simulink model "AFC_FFNN_trainscg_15_15_15_15_15_Nor_July_15_RepCont"  (R2021a)
settings: Solver=ode15s  StartTime=0.0  StopTime=T  MaxStep=.01  RelTol=1e-3
InitFcn:
  | ensure_patch_sig_in();
undefined symbols (not defined in the file): AF_sensor_tol, fault_time, fuel_inj_tol, kappa_tol, MAF_sensor_tol, pump_tol, tau_ww_tol, x_gain, x_offset, y_gain, y_offset
libraries: neural x82
(part 3 of 4)

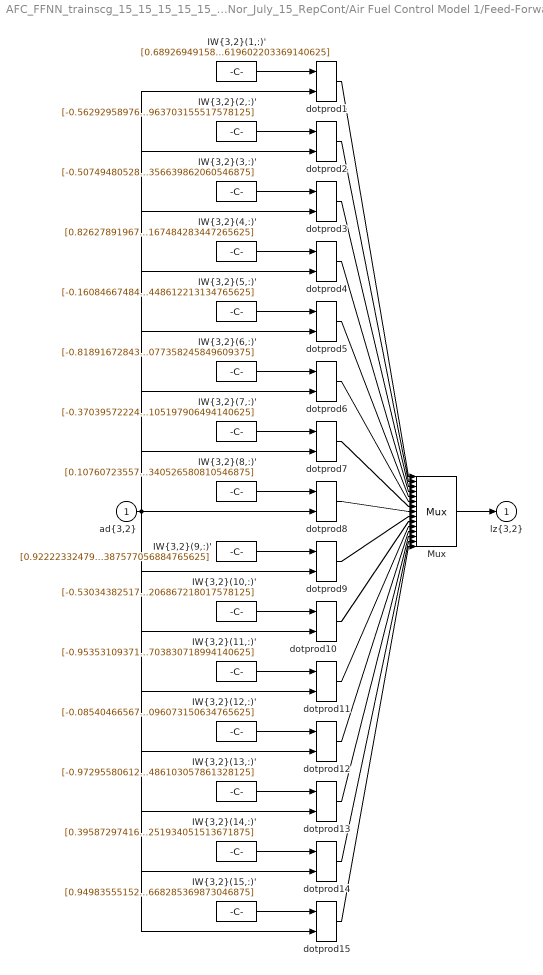
== system AFC_FFNN_trainscg_15_15_15_15_15_Nor_July_15_RepCont/Air Fuel Control Model 1/Feed-Forward Neural Network/Layer 3/LW{3,2} ==
  "ad{3,2}" : Inport  PortDimensions=15
      mask Display: e = 0.06;c1 = [120 230 180]/255;c2 = ([120 230 180]+0)/(256+128);c3 = ([120 230 180]+128)/(256+128);patch([0 1 1 0],[0 0 1 1],c1);patch([0 1 1 1-e 1-e 0+e],[0 0 1 1-e 0+e 0+e],c2);patch([0 0 1 1-e 0+e 0+e],[0 1 1 1-e 1-e 0+e],c3);plot([0 1 1 0 0],[0 0 1 1 0]);
  "IW{3,2}(1,:)'" : Constant  Value=[0.68926949158478090229351664675050415098667144775390625;-0.64905444834060321834812157248961739242076873779296875;0.7831486761913992733497025255928747355937957763671875;-0.61261901862496159765214542858302593231201171875;0.6429042951633501257191483091446571052074432373046875;-0.414752693122203475173392916985903866589069366455078125;-0.0962218095989033628256947849877178668975830078125;-0.670945891090518831134659194503910839557647705078125;0.60892969517095618670055046095512807369232177734375;0.132741198039494523452930252460646443068981170654296875;-0.057600601034548538914581428116434835828840732574462890625;0.486068283333658868183846379906754009425640106201171875;-0.794885979199396519589981835451908409595489501953125;-0.69121066553226617745764315259293653070926666259765625;-0.7117527019887506245510166991152800619602203369140625]
      mask Display: e = 0.06;c1 = [120 150 230]/255;c2 = ([120 150 230]+0)/383;c3 = ([120 150 230]+128)/383;patch([0 1 1 0],[0 0 1 1],c1);patch([0 1 1 1-e 1-e 0+e],[0 0 1 1-e 0+e 0+e],c2);patch([0 0 1 1-e 0+e 0+e],[0 1 1 1-e 1-e 0+e],c3);plot([0 1 1 0 0],[0 0 1 1 0]);disp('weights');
  "IW{3,2}(10,:)'" : Constant  Value=[-0.53034382517854672389745473992661572992801666259765625;0.86697467324738131111416805651970207691192626953125;0.1227983085759849490870010413345880806446075439453125;0.1020682543837800881902921901200897991657257080078125;0.316351772540197029304209763722610659897327423095703125;-0.282980718830822819409576140969875268638134002685546875;-0.00364319955774927706215748912654817104339599609375;0.0611023243564268181415854996885173022747039794921875;-0.4933274183952125468977101263590157032012939453125;-0.192458458377915475612240925329388119280338287353515625;-0.68593701415923480357861308220890350639820098876953125;-0.262855327129308202760427093380712904036045074462890625;-0.8793423223448504355559407485998235642910003662109375;0.51315921379568474325338911512517370283603668212890625;-0.38244919573806601675869387690909206867218017578125]
      mask Display: e = 0.06;c1 = [120 150 230]/255;c2 = ([120 150 230]+0)/383;c3 = ([120 150 230]+128)/383;patch([0 1 1 0],[0 0 1 1],c1);patch([0 1 1 1-e 1-e 0+e],[0 0 1 1-e 0+e 0+e],c2);patch([0 0 1 1-e 0+e 0+e],[0 1 1 1-e 1-e 0+e],c3);plot([0 1 1 0 0],[0 0 1 1 0]);disp('weights');
  "IW{3,2}(11,:)'" : Constant  Value=[-0.95353109371107824809854491832084022462368011474609375;-0.0106801252669140971096606307355614262633025646209716796875;-0.13341806801815270233646515407599508762359619140625;0.9189527235657564130377750188927166163921356201171875;-0.71682661094343114172033892828039824962615966796875;-0.444461641217060776654079745640046894550323486328125;0.212257352710709223941876189201138913631439208984375;-0.9327321645290667095906655958970077335834503173828125;-0.05127212985187412641607807017862796783447265625;-0.7195320830771059217312313194270245730876922607421875;0.95557244312461409041503657135763205587863922119140625;-0.84607443827369011035699486455996520817279815673828125;0.5912676567652963566246171467355452477931976318359375;-0.4259251297044659434476443493622355163097381591796875;0.1932521141071052994675483205355703830718994140625]
      mask Display: e = 0.06;c1 = [120 150 230]/255;c2 = ([120 150 230]+0)/383;c3 = ([120 150 230]+128)/383;patch([0 1 1 0],[0 0 1 1],c1);patch([0 1 1 1-e 1-e 0+e],[0 0 1 1-e 0+e 0+e],c2);patch([0 0 1 1-e 0+e 0+e],[0 1 1 1-e 1-e 0+e],c3);plot([0 1 1 0 0],[0 0 1 1 0]);disp('weights');
  "IW{3,2}(12,:)'" : Constant  Value=[-0.0854046656743794319055496089276857674121856689453125;-0.0516975049611743120436813114793039858341217041015625;0.6786291324143771674926028936170041561126708984375;0.99883997819401049156340377521701157093048095703125;-0.9424632651980908715216855853213928639888763427734375;-0.1453470674596208933593288747943006455898284912109375;-0.7388862796930426579677941845147870481014251708984375;0.981669669379983123036481629242189228534698486328125;0.8675045904703189147966213567997328937053680419921875;0.0739123875832008447872567558079026639461517333984375;-0.5176211250662430263247415496152825653553009033203125;-0.9231613363171853325894744557444937527179718017578125;0.1173255985049836969125180985429324209690093994140625;-0.9587271311368128490215667625307105481624603271484375;-0.7137937826656772788425087128416635096073150634765625]
      mask Display: e = 0.06;c1 = [120 150 230]/255;c2 = ([120 150 230]+0)/383;c3 = ([120 150 230]+128)/383;patch([0 1 1 0],[0 0 1 1],c1);patch([0 1 1 1-e 1-e 0+e],[0 0 1 1-e 0+e 0+e],c2);patch([0 0 1 1-e 0+e 0+e],[0 1 1 1-e 1-e 0+e],c3);plot([0 1 1 0 0],[0 0 1 1 0]);disp('weights');
  "IW{3,2}(13,:)'" : Constant  Value=[-0.9729558061272209901204632842564024031162261962890625;0.148019201281444134910003640470677055418491363525390625;-0.9601201263948049291485631329123862087726593017578125;-0.457150030592506084747839167903293855488300323486328125;0.881381558568999690095324694993905723094940185546875;-0.578115263594495498722380943945609033107757568359375;-0.5573231148004509361015834656427614390850067138671875;-0.4634683435141138119206516421400010585784912109375;-0.0261862264098524644140297823469154536724090576171875;-0.98366029135030164098907334846444427967071533203125;0.9100587127389923036702157332911156117916107177734375;-0.60658409367462218231281667613075114786624908447265625;0.5397436102716650641042406277847476303577423095703125;-0.70489583483044404577100294773117639124393463134765625;0.3715703476170262309352665397454984486103057861328125]
      mask Display: e = 0.06;c1 = [120 150 230]/255;c2 = ([120 150 230]+0)/383;c3 = ([120 150 230]+128)/383;patch([0 1 1 0],[0 0 1 1],c1);patch([0 1 1 1-e 1-e 0+e],[0 0 1 1-e 0+e 0+e],c2);patch([0 0 1 1-e 0+e 0+e],[0 1 1 1-e 1-e 0+e],c3);plot([0 1 1 0 0],[0 0 1 1 0]);disp('weights');
  "IW{3,2}(14,:)'" : Constant  Value=[0.395872974169953817380473992670886218547821044921875;-0.98742185604539167709248204118921421468257904052734375;0.5005797930699971143297943854122422635555267333984375;0.64459120988025608856020198800251819193363189697265625;0.356616175530686307926231393139460124075412750244140625;0.494785064932234119883247558391303755342960357666015625;-0.7257076431667683902304588627885095775127410888671875;0.7573612430550138441276430967263877391815185546875;0.3588984204049230353206212384975515305995941162109375;0.78325236876618908876679370223428122699260711669921875;0.95428037897558570801237465275335125625133514404296875;-0.10244648072712657371763356195515370927751064300537109375;-0.75263446557823865390446371748112142086029052734375;0.663464732529429834784195918473415076732635498046875;-0.9551689522931325893040366281638853251934051513671875]
      mask Display: e = 0.06;c1 = [120 150 230]/255;c2 = ([120 150 230]+0)/383;c3 = ([120 150 230]+128)/383;patch([0 1 1 0],[0 0 1 1],c1);patch([0 1 1 1-e 1-e 0+e],[0 0 1 1-e 0+e 0+e],c2);patch([0 0 1 1-e 0+e 0+e],[0 1 1 1-e 1-e 0+e],c3);plot([0 1 1 0 0],[0 0 1 1 0]);disp('weights');
  "IW{3,2}(15,:)'" : Constant  Value=[0.9498355515277545624286403835867531597614288330078125;-0.1717845436227796174222248737351037561893463134765625;-0.0778938048783024417076603640452958643436431884765625;0.7986556359639991331533792617847211658954620361328125;-0.21212020938234577016601178911514580249786376953125;-0.951507249067342630866050967597402632236480712890625;-0.266562281207658458015430369414389133453369140625;0.1347170460220714627297411425388418138027191162109375;-0.8966633298562920462160263923578895628452301025390625;0.72298581510557990981169496080838143825531005859375;-0.4486463814792076565396428122767247259616851806640625;-0.4543897029028460821109547396190464496612548828125;0.75523401470857454143015274894423782825469970703125;0.3762590257581537311892816433100961148738861083984375;-0.4430234290704671007432580154272727668285369873046875]
      mask Display: e = 0.06;c1 = [120 150 230]/255;c2 = ([120 150 230]+0)/383;c3 = ([120 150 230]+128)/383;patch([0 1 1 0],[0 0 1 1],c1);patch([0 1 1 1-e 1-e 0+e],[0 0 1 1-e 0+e 0+e],c2);patch([0 0 1 1-e 0+e 0+e],[0 1 1 1-e 1-e 0+e],c3);plot([0 1 1 0 0],[0 0 1 1 0]);disp('weights');
  "IW{3,2}(2,:)'" : Constant  Value=[-0.562929589768697002938324658316560089588165283203125;0.165651753034273152564992415136657655239105224609375;0.9568583771587524378077205255976878106594085693359375;0.5560316320103704246236020480864681303501129150390625;-0.238504282118257027178742646356113255023956298828125;0.8005401741912212543184068636037409305572509765625;-0.93901775570367806977856162120588123798370361328125;-0.688989783220818718945110958884470164775848388671875;-0.9128197821751562468506335790152661502361297607421875;-0.763621831076356283318773421342484652996063232421875;-0.935670688003623407524855792871676385402679443359375;-0.68908866271854751772707459167577326297760009765625;-0.269619161332864454294622191810049116611480712890625;0.9672060355241896001388113290886394679546356201171875;-0.0859138894842665923334834587876684963703155517578125]
      mask Display: e = 0.06;c1 = [120 150 230]/255;c2 = ([120 150 230]+0)/383;c3 = ([120 150 230]+128)/383;patch([0 1 1 0],[0 0 1 1],c1);patch([0 1 1 1-e 1-e 0+e],[0 0 1 1-e 0+e 0+e],c2);patch([0 0 1 1-e 0+e 0+e],[0 1 1 1-e 1-e 0+e],c3);plot([0 1 1 0 0],[0 0 1 1 0]);disp('weights');
  "IW{3,2}(3,:)'" : Constant  Value=[-0.5074948052874506121412423453875817358493804931640625;0.77053787988654953711176176511798985302448272705078125;-0.7363382298223342115051082146237604320049285888671875;0.78742202814315975789583035293617285788059234619140625;0.52418306688785365476945798945962451398372650146484375;0.0303079115437369962793301425563186057843267917633056640625;-0.68992151593302697420995173160918056964874267578125;-0.2673862720881918786375308627611957490444183349609375;0.1387208230034355782578359139733947813510894775390625;-0.0227437019702670210896666702637958223931491374969482421875;-0.7903579986247384336905952295637689530849456787109375;-0.71092558778322756385392722222604788839817047119140625;-0.85751150675600040784729571896605193614959716796875;0.66081167614687874589662897051312029361724853515625;-0.4849577362305506067485794119420461356639862060546875]
      mask Display: e = 0.06;c1 = [120 150 230]/255;c2 = ([120 150 230]+0)/383;c3 = ([120 150 230]+128)/383;patch([0 1 1 0],[0 0 1 1],c1);patch([0 1 1 1-e 1-e 0+e],[0 0 1 1-e 0+e 0+e],c2);patch([0 0 1 1-e 0+e 0+e],[0 1 1 1-e 1-e 0+e],c3);plot([0 1 1 0 0],[0 0 1 1 0]);disp('weights');
  "IW{3,2}(4,:)'" : Constant  Value=[0.8262789196706921135415768731036223471164703369140625;0.7796907145922069570787016346002928912639617919921875;0.863358666186659906571776446071453392505645751953125;0.2554357997803824442684117457247339189052581787109375;0.77856833338737863048351073302910663187503814697265625;0.349985156215272985580355680212960578501224517822265625;0.8537423607916221346414431536686606705188751220703125;-0.131939451533888973955299661611206829547882080078125;0.169808359894214166985193514847196638584136962890625;0.2302788227858534597647377495377440936863422393798828125;-0.87119703430520767373224089169525541365146636962890625;0.5464001123132897763667870094650425016880035400390625;0.07753581185590530111539919744245707988739013671875;0.5963829717247104422739312212797813117504119873046875;-0.2857582500055375618330799625255167484283447265625]
      mask Display: e = 0.06;c1 = [120 150 230]/255;c2 = ([120 150 230]+0)/383;c3 = ([120 150 230]+128)/383;patch([0 1 1 0],[0 0 1 1],c1);patch([0 1 1 1-e 1-e 0+e],[0 0 1 1-e 0+e 0+e],c2);patch([0 0 1 1-e 0+e 0+e],[0 1 1 1-e 1-e 0+e],c3);plot([0 1 1 0 0],[0 0 1 1 0]);disp('weights');
  "IW{3,2}(5,:)'" : Constant  Value=[-0.160846674847559878429592572501860558986663818359375;0.5725155963220462940199695367482490837574005126953125;-0.983765381681773742883478917065076529979705810546875;0.9883897465709858831672818268998526036739349365234375;-0.046437458085572487498371430092447553761303424835205078125;-0.8774053710440583575547179862041957676410675048828125;0.3322310252958544651846750639379024505615234375;-0.4657403300045681593388735564076341688632965087890625;0.123325125465898910448458991595543920993804931640625;0.732605515826929565292857660097070038318634033203125;-0.09622216208059765352178516195635893382132053375244140625;-0.90586018869653706087063937957282178103923797607421875;-0.92720323014644545622786608873866498470306396484375;-0.02650061922837831929200547165237367153167724609375;-0.0226346575634099878016058937646448612213134765625]
      mask Display: e = 0.06;c1 = [120 150 230]/255;c2 = ([120 150 230]+0)/383;c3 = ([120 150 230]+128)/383;patch([0 1 1 0],[0 0 1 1],c1);patch([0 1 1 1-e 1-e 0+e],[0 0 1 1-e 0+e 0+e],c2);patch([0 0 1 1-e 0+e 0+e],[0 1 1 1-e 1-e 0+e],c3);plot([0 1 1 0 0],[0 0 1 1 0]);disp('weights');
  "IW{3,2}(6,:)'" : Constant  Value=[-0.8189167284368645827186128371977247297763824462890625;0.061807328063784527927282397286035120487213134765625;0.017844064952306393223580016638152301311492919921875;-0.9692901124822135283665147653664462268352508544921875;-0.0650675268659763883505320336553268134593963623046875;-0.66108982877411648360066465102136135101318359375;0.6150896999685613319996946302126161754131317138671875;-0.9475317479734639558586195562384091317653656005859375;0.27864289333406677684479291201569139957427978515625;-0.0999710377048177445402643570560030639171600341796875;0.255282171335795116107192370691336691379547119140625;0.02957999373653930064165251678787171840667724609375;0.883203184300609844825658001354895532131195068359375;-0.948810814237413868710291353636421263217926025390625;-0.3728712112794771993407039190060459077358245849609375]
      mask Display: e = 0.06;c1 = [120 150 230]/255;c2 = ([120 150 230]+0)/383;c3 = ([120 150 230]+128)/383;patch([0 1 1 0],[0 0 1 1],c1);patch([0 1 1 1-e 1-e 0+e],[0 0 1 1-e 0+e 0+e],c2);patch([0 0 1 1-e 0+e 0+e],[0 1 1 1-e 1-e 0+e],c3);plot([0 1 1 0 0],[0 0 1 1 0]);disp('weights');
  "IW{3,2}(7,:)'" : Constant  Value=[-0.370395722246221359430506936405436135828495025634765625;0.044590764100431772021249088311378727667033672332763671875;0.8785175341474076304848495055921375751495361328125;-0.976943983770184321002716387738473713397979736328125;0.43236263507675920525485935286269523203372955322265625;-0.296324961438232670207781893623177893459796905517578125;-0.789793825881249578202414340921677649021148681640625;0.5878218515385345011026174688595347106456756591796875;0.2276506223106313786530563447740860283374786376953125;-0.28010679864059684351929035983630456030368804931640625;-0.5399230455464418820810124088893644511699676513671875;0.6545030236788258459768030661507509648799896240234375;0.65644071566094197578422608785331249237060546875;0.322146894332130229177124647321761585772037506103515625;0.8296626813005973932746428545215167105197906494140625]
      mask Display: e = 0.06;c1 = [120 150 230]/255;c2 = ([120 150 230]+0)/383;c3 = ([120 150 230]+128)/383;patch([0 1 1 0],[0 0 1 1],c1);patch([0 1 1 1-e 1-e 0+e],[0 0 1 1-e 0+e 0+e],c2);patch([0 0 1 1-e 0+e 0+e],[0 1 1 1-e 1-e 0+e],c3);plot([0 1 1 0 0],[0 0 1 1 0]);disp('weights');
  "IW{3,2}(8,:)'" : Constant  Value=[0.1076072355737454355750770673694205470383167266845703125;0.431186084387213564017571343356394208967685699462890625;0.9569188082777533299605465799686498939990997314453125;0.357552931921336913934084122956846840679645538330078125;-0.335665225712111381373148333295830525457859039306640625;0.301799808964890281526294302238966338336467742919921875;0.032457440638200996119167029974050819873809814453125;-0.86921450426542801181994946091435849666595458984375;0.6065302952189728369347676562028937041759490966796875;0.33424202847897721557757222399231977760791778564453125;-0.09915225011524893272696346002703648991882801055908203125;0.59735452974551439542238995272782631218433380126953125;-0.9641615996222643314439437745022587478160858154296875;0.34897273551590035634006881082314066588878631591796875;-0.4773999403397606311472145534935407340526580810546875]
      mask Display: e = 0.06;c1 = [120 150 230]/255;c2 = ([120 150 230]+0)/383;c3 = ([120 150 230]+128)/383;patch([0 1 1 0],[0 0 1 1],c1);patch([0 1 1 1-e 1-e 0+e],[0 0 1 1-e 0+e 0+e],c2);patch([0 0 1 1-e 0+e 0+e],[0 1 1 1-e 1-e 0+e],c3);plot([0 1 1 0 0],[0 0 1 1 0]);disp('weights');
  "IW{3,2}(9,:)'" : Constant  Value=[0.9222233247908968589712230823352001607418060302734375;-0.9651347018682070455497523653320968151092529296875;0.3126439464082562125213371473364531993865966796875;0.05283618341942375451480984338559210300445556640625;-0.278834754216143121396953574731014668941497802734375;-0.64437479507781869614291281322948634624481201171875;-0.975672238166819472127144763362593948841094970703125;0.1307382086248607411249622600735165178775787353515625;-0.1294502888130011353240433891187421977519989013671875;-0.634352160035149825745293128420598804950714111328125;-0.8981519511431492741593274331535212695598602294921875;-0.318787575353978613890149063081480562686920166015625;-0.4154144334619822576115666379337199032306671142578125;-0.465902387041180698901143841794691979885101318359375;-0.3111476799713577268136077691451646387577056884765625]
      mask Display: e = 0.06;c1 = [120 150 230]/255;c2 = ([120 150 230]+0)/383;c3 = ([120 150 230]+128)/383;patch([0 1 1 0],[0 0 1 1],c1);patch([0 1 1 1-e 1-e 0+e],[0 0 1 1-e 0+e 0+e],c2);patch([0 0 1 1-e 0+e 0+e],[0 1 1 1-e 1-e 0+e],c3);plot([0 1 1 0 0],[0 0 1 1 0]);disp('weights');
  Mux : Mux  Inputs=15
      mask Display: e = 0.06;c1 = [120 150 230]/255;c2 = ([120 150 230]+0)/383;c3 = ([120 150 230]+128)/383;patch([0 1 1 0],[0 0 1 1],c1);patch([0 1 1 1-e 1-e 0+e],[0 0 1 1-e 0+e 0+e],c2);patch([0 0 1 1-e 0+e 0+e],[0 1 1 1-e 1-e 0+e],c3);plot([0 1 1 0 0],[0 0 1 1 0]);disp('Mux');
  dotprod{1..15} (15 alike) : neural/Weight Functions/dotprod
  "lz{3,2}" : Outport
      mask Display: e = 0.06;c1 = [120 230 180]/255;c2 = ([120 230 180]+0)/(256+128);c3 = ([120 230 180]+128)/(256+128);patch([0 1 1 0],[0 0 1 1],c1);patch([0 1 1 1-e 1-e 0+e],[0 0 1 1-e 0+e 0+e],c2);patch([0 0 1 1-e 0+e 0+e],[0 1 1 1-e 1-e 0+e],c3);plot([0 1 1 0 0],[0 0 1 1 0]);
  wires:
  Mux/1 -> "lz{3,2}"/1
  dotprod15/1 -> Mux/15
  "IW{3,2}(15,:)'"/1 -> dotprod15/1
  dotprod14/1 -> Mux/14
  "IW{3,2}(14,:)'"/1 -> dotprod14/1
  dotprod13/1 -> Mux/13
  "IW{3,2}(13,:)'"/1 -> dotprod13/1
  dotprod12/1 -> Mux/12
  "IW{3,2}(12,:)'"/1 -> dotprod12/1
  dotprod11/1 -> Mux/11
  "IW{3,2}(11,:)'"/1 -> dotprod11/1
  dotprod10/1 -> Mux/10
  "IW{3,2}(10,:)'"/1 -> dotprod10/1
  dotprod9/1 -> Mux/9
  "IW{3,2}(9,:)'"/1 -> dotprod9/1
  dotprod8/1 -> Mux/8
  "IW{3,2}(8,:)'"/1 -> dotprod8/1
  dotprod7/1 -> Mux/7
  "IW{3,2}(7,:)'"/1 -> dotprod7/1
  dotprod6/1 -> Mux/6
  "IW{3,2}(6,:)'"/1 -> dotprod6/1
  dotprod5/1 -> Mux/5
  "IW{3,2}(5,:)'"/1 -> dotprod5/1
  dotprod4/1 -> Mux/4
  "IW{3,2}(4,:)'"/1 -> dotprod4/1
  dotprod3/1 -> Mux/3
  "IW{3,2}(3,:)'"/1 -> dotprod3/1
  dotprod2/1 -> Mux/2
  "IW{3,2}(2,:)'"/1 -> dotprod2/1
  dotprod1/1 -> Mux/1
  "ad{3,2}"/1 -> dotprod15/2, dotprod14/2, dotprod13/2, dotprod12/2, dotprod11/2, dotprod10/2, dotprod9/2, dotprod8/2, dotprod7/2, dotprod6/2, dotprod5/2, dotprod4/2, dotprod3/2, dotprod2/2, dotprod1/2
  "IW{3,2}(1,:)'"/1 -> dotprod1/1

== system AFC_FFNN_trainscg_15_15_15_15_15_Nor_July_15_RepCont/Air Fuel Control Model 1/Feed-Forward Neural Network/Layer 4/Delays 1 ==
  "p{4}" : Inport  PortDimensions=15
      mask Display: e = 0.06;c1 = [120 230 180]/255;c2 = ([120 230 180]+0)/(256+128);c3 = ([120 230 180]+128)/(256+128);patch([0 1 1 0],[0 0 1 1],c1);patch([0 1 1 1-e 1-e 0+e],[0 0 1 1-e 0+e 0+e],c2);patch([0 0 1 1-e 0+e 0+e],[0 1 1 1-e 1-e 0+e],c3);plot([0 1 1 0 0],[0 0 1 1 0]);
  mux : Mux  Inputs=1
      mask Display: e = 0.06;c1 = [120 150 230]/255;c2 = ([120 150 230]+0)/383;c3 = ([120 150 230]+128)/383;patch([0 1 1 0],[0 0 1 1],c1);patch([0 1 1 1-e 1-e 0+e],[0 0 1 1-e 0+e 0+e],c2);patch([0 0 1 1-e 0+e 0+e],[0 1 1 1-e 1-e 0+e],c3);plot([0 1 1 0 0],[0 0 1 1 0]);disp('Mux')
  "pd{4,3}" : Outport
      mask Display: e = 0.06;c1 = [120 230 180]/255;c2 = ([120 230 180]+0)/(256+128);c3 = ([120 230 180]+128)/(256+128);patch([0 1 1 0],[0 0 1 1],c1);patch([0 1 1 1-e 1-e 0+e],[0 0 1 1-e 0+e 0+e],c2);patch([0 0 1 1-e 0+e 0+e],[0 1 1 1-e 1-e 0+e],c3);plot([0 1 1 0 0],[0 0 1 1 0]);
  wires:
  mux/1 -> "pd{4,3}"/1
  "p{4}"/1 -> mux/1

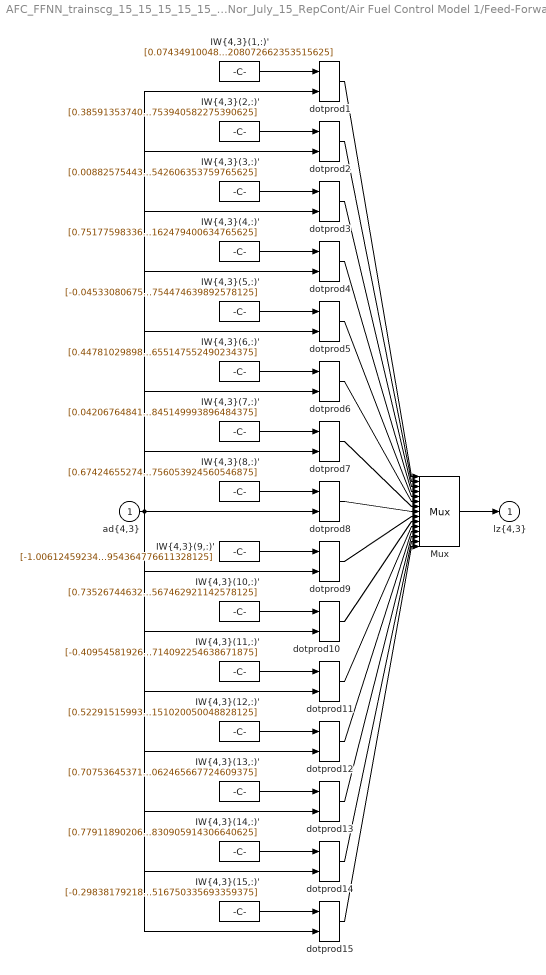
== system AFC_FFNN_trainscg_15_15_15_15_15_Nor_July_15_RepCont/Air Fuel Control Model 1/Feed-Forward Neural Network/Layer 4/LW{4,3} ==
  "ad{4,3}" : Inport  PortDimensions=15
      mask Display: e = 0.06;c1 = [120 230 180]/255;c2 = ([120 230 180]+0)/(256+128);c3 = ([120 230 180]+128)/(256+128);patch([0 1 1 0],[0 0 1 1],c1);patch([0 1 1 1-e 1-e 0+e],[0 0 1 1-e 0+e 0+e],c2);patch([0 0 1 1-e 0+e 0+e],[0 1 1 1-e 1-e 0+e],c3);plot([0 1 1 0 0],[0 0 1 1 0]);
  "IW{4,3}(1,:)'" : Constant  Value=[0.074349100483344032763710629296838305890560150146484375;-0.2325662791511675653310931011219508945941925048828125;-0.5381154884542291849669481962337158620357513427734375;0.1386295109502034550441607052562176249921321868896484375;-0.37797625642184240479792833866667933762073516845703125;0.6500953139118197388057751595624722540378570556640625;-0.71645051950191429579462010224233381450176239013671875;-0.42415904949149141334174828443792648613452911376953125;-0.522087717682781171646411166875623166561126708984375;0.2134427609428042327266439315280877053737640380859375;-0.9265960947882854181756329126073978841304779052734375;-0.1461549422446244417272964710718952119350433349609375;0.496156728707464911298785636972752399742603302001953125;-0.467980089049811087686947530528414063155651092529296875;-0.828161988219234590502537685097195208072662353515625]
      mask Display: e = 0.06;c1 = [120 150 230]/255;c2 = ([120 150 230]+0)/383;c3 = ([120 150 230]+128)/383;patch([0 1 1 0],[0 0 1 1],c1);patch([0 1 1 1-e 1-e 0+e],[0 0 1 1-e 0+e 0+e],c2);patch([0 0 1 1-e 0+e 0+e],[0 1 1 1-e 1-e 0+e],c3);plot([0 1 1 0 0],[0 0 1 1 0]);disp('weights');
  "IW{4,3}(10,:)'" : Constant  Value=[0.7352674463222312883914355552406050264835357666015625;-0.6220688627615544863402874398161657154560089111328125;-0.4612868378094046040160947086405940353870391845703125;-0.7690744341636996939115533677977509796619415283203125;0.364523315808154446671096593490801751613616943359375;-0.5505544008294369628941922201192937791347503662109375;0.9440421013235733571633545579970814287662506103515625;-0.2344205461328694450884313482674770057201385498046875;-0.3421493061719094175288091719266958534717559814453125;-0.7250516891389173768089904115186072885990142822265625;-0.2911601662961176284483144627301953732967376708984375;0.4865548552326515174826226939330808818340301513671875;-0.614256005760669854254274468985386192798614501953125;-0.14911166211352355759345300612039864063262939453125;0.9353193529802219519098116506938822567462921142578125]
      mask Display: e = 0.06;c1 = [120 150 230]/255;c2 = ([120 150 230]+0)/383;c3 = ([120 150 230]+128)/383;patch([0 1 1 0],[0 0 1 1],c1);patch([0 1 1 1-e 1-e 0+e],[0 0 1 1-e 0+e 0+e],c2);patch([0 0 1 1-e 0+e 0+e],[0 1 1 1-e 1-e 0+e],c3);plot([0 1 1 0 0],[0 0 1 1 0]);disp('weights');
  "IW{4,3}(11,:)'" : Constant  Value=[-0.40954581926718258699793295818381011486053466796875;-0.209952151050021740275042247958481311798095703125;-0.2064904433647580805910592971486039459705352783203125;0.1238876984131753733464620381710119545459747314453125;0.2207973745056917014295549961389042437076568603515625;0.4043229885403072376703903501038439571857452392578125;0.16052297693793082800084448535926640033721923828125;-0.1510627772562316284421513046254403889179229736328125;0.625340446388026105495328010874800384044647216796875;-0.737940333490474387190261040814220905303955078125;-0.081506414055812381747045947122387588024139404296875;0.5640702366617400542736504576168954372406005859375;-0.1445523819865301984322059070109389722347259521484375;-0.573360915257262515609681940986774861812591552734375;0.36503182909853659765531119774095714092254638671875]
      mask Display: e = 0.06;c1 = [120 150 230]/255;c2 = ([120 150 230]+0)/383;c3 = ([120 150 230]+128)/383;patch([0 1 1 0],[0 0 1 1],c1);patch([0 1 1 1-e 1-e 0+e],[0 0 1 1-e 0+e 0+e],c2);patch([0 0 1 1-e 0+e 0+e],[0 1 1 1-e 1-e 0+e],c3);plot([0 1 1 0 0],[0 0 1 1 0]);disp('weights');
  "IW{4,3}(12,:)'" : Constant  Value=[0.5229151599398147443054085670155473053455352783203125;0.0668062429593738738020647360826842486858367919921875;0.10388454329580172619262867783618276007473468780517578125;-0.6445508987129973110796754554030485451221466064453125;0.10760557398696679598515402176417410373687744140625;-0.8975738027855137968202825504704378545284271240234375;0.4048106195281306884936611822922714054584503173828125;0.7646290355386236026191681958152912557125091552734375;0.808722577754244387193693910376168787479400634765625;-0.369588474634115815575796659686602652072906494140625;0.927177911226604312133758867275901138782501220703125;0.2464285148358735799689611667417921125888824462890625;-0.7710168032929891612781148069188930094242095947265625;0.9789119736813682859377649947418831288814544677734375;-0.4766114794815010657913489922066219151020050048828125]
      mask Display: e = 0.06;c1 = [120 150 230]/255;c2 = ([120 150 230]+0)/383;c3 = ([120 150 230]+128)/383;patch([0 1 1 0],[0 0 1 1],c1);patch([0 1 1 1-e 1-e 0+e],[0 0 1 1-e 0+e 0+e],c2);patch([0 0 1 1-e 0+e 0+e],[0 1 1 1-e 1-e 0+e],c3);plot([0 1 1 0 0],[0 0 1 1 0]);disp('weights');
  "IW{4,3}(13,:)'" : Constant  Value=[0.7075364537119337438042521171155385673046112060546875;-0.767668879818697913464120574644766747951507568359375;0.55007147010354884297811395299504511058330535888671875;-0.6106701140328276711244370744680054485797882080078125;0.6972476042524231587549365940503776073455810546875;-0.5354868194475292941802990753785707056522369384765625;0.76167148072680157522285071536316536366939544677734375;-0.42180889329320836456105325851240195333957672119140625;0.7665122361950833518307035774341784417629241943359375;0.90348869713702295580759482618304900825023651123046875;-0.07351895802781971411832273588515818119049072265625;-0.32664730128458874247598942019976675510406494140625;0.6420791870935589340518845347105525434017181396484375;0.74761179512886855036413180641829967498779296875;0.0630118524273972635540985720581375062465667724609375]
      mask Display: e = 0.06;c1 = [120 150 230]/255;c2 = ([120 150 230]+0)/383;c3 = ([120 150 230]+128)/383;patch([0 1 1 0],[0 0 1 1],c1);patch([0 1 1 1-e 1-e 0+e],[0 0 1 1-e 0+e 0+e],c2);patch([0 0 1 1-e 0+e 0+e],[0 1 1 1-e 1-e 0+e],c3);plot([0 1 1 0 0],[0 0 1 1 0]);disp('weights');
  "IW{4,3}(14,:)'" : Constant  Value=[0.77911890206766043487363049280247651040554046630859375;0.3005314436787875909118383788154460489749908447265625;-0.54636206669537357161203772193402983248233795166015625;0.9024541534967465139516207273118197917938232421875;-0.4392096744089373228092654244392178952693939208984375;0.8217256204724023849195191360195167362689971923828125;-0.85371688118925115329460595603450201451778411865234375;0.9714487780644256442741379942162893712520599365234375;-0.324928767306938315329034594469703733921051025390625;-0.18058611694917792167558445726172067224979400634765625;-0.49537725304021062999737523568910546600818634033203125;0.263288327783642639445815802901051938533782958984375;-0.78974407950721126070448008249513804912567138671875;-0.1353463946125611216952933091306476853787899017333984375;-0.76662709328578504397455617436207830905914306640625]
      mask Display: e = 0.06;c1 = [120 150 230]/255;c2 = ([120 150 230]+0)/383;c3 = ([120 150 230]+128)/383;patch([0 1 1 0],[0 0 1 1],c1);patch([0 1 1 1-e 1-e 0+e],[0 0 1 1-e 0+e 0+e],c2);patch([0 0 1 1-e 0+e 0+e],[0 1 1 1-e 1-e 0+e],c3);plot([0 1 1 0 0],[0 0 1 1 0]);disp('weights');
  "IW{4,3}(15,:)'" : Constant  Value=[-0.29838179218397942182861015680828131735324859619140625;-0.37980098378279070203689116169698536396026611328125;-0.713707971537280716489703991101123392581939697265625;0.64570511445325584620746894870535470545291900634765625;0.66287395927729686473384163036826066672801971435546875;0.7270563419832811735687982945819385349750518798828125;-0.80988272704156150094689792240387760102748870849609375;-0.385462680469129070903733236264088191092014312744140625;0.5320320191253158359501185259432531893253326416015625;-0.83917312760953965966592704717186279594898223876953125;0.475406841289294834762557684371131472289562225341796875;-0.577934513428964624637274027918465435504913330078125;0.75053184919748339165579409382189624011516571044921875;-0.38820027172205839871566013243864290416240692138671875;0.5454486372483839939917515948764048516750335693359375]
      mask Display: e = 0.06;c1 = [120 150 230]/255;c2 = ([120 150 230]+0)/383;c3 = ([120 150 230]+128)/383;patch([0 1 1 0],[0 0 1 1],c1);patch([0 1 1 1-e 1-e 0+e],[0 0 1 1-e 0+e 0+e],c2);patch([0 0 1 1-e 0+e 0+e],[0 1 1 1-e 1-e 0+e],c3);plot([0 1 1 0 0],[0 0 1 1 0]);disp('weights');
  "IW{4,3}(2,:)'" : Constant  Value=[0.3859135374030469023409750661812722682952880859375;-0.4894480863430576977890495982137508690357208251953125;-0.8142243049217905426218067077570594847202301025390625;0.26351365588004604934013741512899287045001983642578125;-0.4254725573061353127712891364353708922863006591796875;0.4245532726916321220045347217819653451442718505859375;-0.53889807056561778164649467726121656596660614013671875;-0.86653218037656942751567612504004500806331634521484375;-0.9077254461771564475469631361193023622035980224609375;-0.2742643448700714525756438888492994010448455810546875;0.9801391081252024406467171502299606800079345703125;0.4004532154034503577122450224123895168304443359375;-0.515123397728948884122246454353444278240203857421875;0.83948484916209864525882267116685397922992706298828125;-0.2404448709700057751348367673926986753940582275390625]
      mask Display: e = 0.06;c1 = [120 150 230]/255;c2 = ([120 150 230]+0)/383;c3 = ([120 150 230]+128)/383;patch([0 1 1 0],[0 0 1 1],c1);patch([0 1 1 1-e 1-e 0+e],[0 0 1 1-e 0+e 0+e],c2);patch([0 0 1 1-e 0+e 0+e],[0 1 1 1-e 1-e 0+e],c3);plot([0 1 1 0 0],[0 0 1 1 0]);disp('weights');
  "IW{4,3}(3,:)'" : Constant  Value=[0.00882575443026384874600775987119050114415585994720458984375;-0.062257512940821602143159907427616417407989501953125;0.22176632576290800091811661332030780613422393798828125;0.98680076580737752234284698715782724320888519287109375;0.548050180662683406040969202877022325992584228515625;0.055703066312880356036885132198221981525421142578125;-0.17648508211840396864289459699648432433605194091796875;-0.6791773543076959906983347536879591643810272216796875;0.4688111691864531582751851601642556488513946533203125;0.769869284454610891543779871426522731781005859375;-0.0161893332077034900196021993679096340201795101165771484375;0.6909627908365791881806217133998870849609375;-0.83942374213210302347221158925094641745090484619140625;-0.447167619543548777727437482099048793315887451171875;0.25712671417844124022167306975461542606353759765625]
      mask Display: e = 0.06;c1 = [120 150 230]/255;c2 = ([120 150 230]+0)/383;c3 = ([120 150 230]+128)/383;patch([0 1 1 0],[0 0 1 1],c1);patch([0 1 1 1-e 1-e 0+e],[0 0 1 1-e 0+e 0+e],c2);patch([0 0 1 1-e 0+e 0+e],[0 1 1 1-e 1-e 0+e],c3);plot([0 1 1 0 0],[0 0 1 1 0]);disp('weights');
  "IW{4,3}(4,:)'" : Constant  Value=[0.75177598336575979232065947144292294979095458984375;0.3702895784867925588201842401758767664432525634765625;0.8695032651792422573322483003721572458744049072265625;-0.73114286494634683766236094015766866505146026611328125;-0.821469165834722847563398318015970289707183837890625;-0.860110086194837197837159692426212131977081298828125;-0.98228400009632166334228031701059080660343170166015625;0.17978824004549542880937451627687551081180572509765625;0.619843911574649464313324642716906964778900146484375;0.2170230000325425734342132955134729854762554168701171875;0.5392351431665025618400477469549514353275299072265625;-0.6687457292709984013612256603664718568325042724609375;0.59422170211557101549004755725036375224590301513671875;-0.70772343920246283399677622583112679421901702880859375;-0.15785270237549386962427888647653162479400634765625]
      mask Display: e = 0.06;c1 = [120 150 230]/255;c2 = ([120 150 230]+0)/383;c3 = ([120 150 230]+128)/383;patch([0 1 1 0],[0 0 1 1],c1);patch([0 1 1 1-e 1-e 0+e],[0 0 1 1-e 0+e 0+e],c2);patch([0 0 1 1-e 0+e 0+e],[0 1 1 1-e 1-e 0+e],c3);plot([0 1 1 0 0],[0 0 1 1 0]);disp('weights');
  "IW{4,3}(5,:)'" : Constant  Value=[-0.0453308067579560880488998009241186082363128662109375;-0.360452489509979212556345373741351068019866943359375;-0.908340968616638377852723351679742336273193359375;0.4455634035465834141831464876304380595684051513671875;-0.543489712917239131684254971332848072052001953125;-0.7003784462962896473214868819923140108585357666015625;-0.3159000630638961748530846307403407990932464599609375;-0.731838328583773733981843179208226501941680908203125;-0.194505218857061290549381737946532666683197021484375;-0.8204981840788028168987011667923070490360260009765625;0.017976674577256712694861562340520322322845458984375;-0.7393429432134492884642895660363137722015380859375;-0.8947192019853116295990957951289601624011993408203125;-0.502834162304892640094067246536724269390106201171875;-0.0919987924902649911729213272337801754474639892578125]
      mask Display: e = 0.06;c1 = [120 150 230]/255;c2 = ([120 150 230]+0)/383;c3 = ([120 150 230]+128)/383;patch([0 1 1 0],[0 0 1 1],c1);patch([0 1 1 1-e 1-e 0+e],[0 0 1 1-e 0+e 0+e],c2);patch([0 0 1 1-e 0+e 0+e],[0 1 1 1-e 1-e 0+e],c3);plot([0 1 1 0 0],[0 0 1 1 0]);disp('weights');
  "IW{4,3}(6,:)'" : Constant  Value=[0.4478102989897096986027236198424361646175384521484375;-0.791832975254418425237190604093484580516815185546875;-0.27812353995312122378891217522323131561279296875;-0.4752399215035738588852609609602950513362884521484375;0.9418475099537635397695112260407768189907073974609375;0.4676998024269225506799330105422995984554290771484375;-0.683056658237144898038195606204681098461151123046875;0.5205910196036007686615221246029250323772430419921875;-0.8051914277071781089745172721450217068195343017578125;-0.9068754386092916508488315230351872742176055908203125;-0.146768962619944431935437023639678955078125;0.090061692476291366205032318248413503170013427734375;-0.0920349863494422937293393260915763676166534423828125;-0.90089856406488078022221088758669793605804443359375;0.98467304515324283187283072038553655147552490234375]
      mask Display: e = 0.06;c1 = [120 150 230]/255;c2 = ([120 150 230]+0)/383;c3 = ([120 150 230]+128)/383;patch([0 1 1 0],[0 0 1 1],c1);patch([0 1 1 1-e 1-e 0+e],[0 0 1 1-e 0+e 0+e],c2);patch([0 0 1 1-e 0+e 0+e],[0 1 1 1-e 1-e 0+e],c3);plot([0 1 1 0 0],[0 0 1 1 0]);disp('weights');
  "IW{4,3}(7,:)'" : Constant  Value=[0.042067648411856638224204374409964657388627529144287109375;-0.421486373774265121738835659925825893878936767578125;0.343874306823647390984888261300511658191680908203125;0.79461083619435246561124586150981485843658447265625;0.356971966037631094348370197621989063918590545654296875;-0.9032242250105102510104870816576294600963592529296875;-0.7838942367168808544874991639517247676849365234375;-0.450664356120435705133075998674030415713787078857421875;-0.9820753603085534688688085225294344127178192138671875;-0.66608152346287996525830976679571904242038726806640625;0.1910375355868025593064629674699972383677959442138671875;0.55915736478190769531693149474449455738067626953125;0.53949172083467267224676788828219287097454071044921875;-0.81394298977268497718995376999373547732830047607421875;0.4953742466469905902926029739319346845149993896484375]
      mask Display: e = 0.06;c1 = [120 150 230]/255;c2 = ([120 150 230]+0)/383;c3 = ([120 150 230]+128)/383;patch([0 1 1 0],[0 0 1 1],c1);patch([0 1 1 1-e 1-e 0+e],[0 0 1 1-e 0+e 0+e],c2);patch([0 0 1 1-e 0+e 0+e],[0 1 1 1-e 1-e 0+e],c3);plot([0 1 1 0 0],[0 0 1 1 0]);disp('weights');
  "IW{4,3}(8,:)'" : Constant  Value=[0.6742465527460999030751054306165315210819244384765625;-0.899561043625946243906810195767320692539215087890625;-0.78701267863605373076296700673992745578289031982421875;0.769883275579368753227527122362516820430755615234375;-0.67511918761967637525600594017305411398410797119140625;0.724313351342086964024247208726592361927032470703125;-0.6547149468694486440512037006556056439876556396484375;-0.60395776936510336962982137265498749911785125732421875;-0.9805221777048058751091730300686322152614593505859375;-0.303828044108071682050109529882320202887058258056640625;-0.58397388447369491526472984332940541207790374755859375;-0.6918144040871510025425550338695757091045379638671875;-0.56721303386631849452470532924053259193897247314453125;-0.7694745913482907706537616832065396010875701904296875;-0.8864506383956534119050729714217595756053924560546875]
      mask Display: e = 0.06;c1 = [120 150 230]/255;c2 = ([120 150 230]+0)/383;c3 = ([120 150 230]+128)/383;patch([0 1 1 0],[0 0 1 1],c1);patch([0 1 1 1-e 1-e 0+e],[0 0 1 1-e 0+e 0+e],c2);patch([0 0 1 1-e 0+e 0+e],[0 1 1 1-e 1-e 0+e],c3);plot([0 1 1 0 0],[0 0 1 1 0]);disp('weights');
  "IW{4,3}(9,:)'" : Constant  Value=[-1.0061245923459816165035363155766390264034271240234375;-0.6758029107273058055938008692464791238307952880859375;0.57623520196881783395070897313416935503482818603515625;0.1790242759025365282266051281112595461308956146240234375;-0.414272155068949654577181718195788562297821044921875;-0.015310692783815138540148836909793317317962646484375;0.40768868235542032874008100407081656157970428466796875;-0.73169230261350792776653406690456904470920562744140625;-0.494754223084045374747574896900914609432220458984375;0.51022108874891325402955999379628337919712066650390625;-0.3487405101885940883477132956613786518573760986328125;-0.7242981496196378987662001236458308994770050048828125;0.1746445515014139193699094221301493234932422637939453125;-0.11752990942164535936864666609835694544017314910888671875;-0.0952112383005527807000589746166951954364776611328125]
      mask Display: e = 0.06;c1 = [120 150 230]/255;c2 = ([120 150 230]+0)/383;c3 = ([120 150 230]+128)/383;patch([0 1 1 0],[0 0 1 1],c1);patch([0 1 1 1-e 1-e 0+e],[0 0 1 1-e 0+e 0+e],c2);patch([0 0 1 1-e 0+e 0+e],[0 1 1 1-e 1-e 0+e],c3);plot([0 1 1 0 0],[0 0 1 1 0]);disp('weights');
  Mux : Mux  Inputs=15
      mask Display: e = 0.06;c1 = [120 150 230]/255;c2 = ([120 150 230]+0)/383;c3 = ([120 150 230]+128)/383;patch([0 1 1 0],[0 0 1 1],c1);patch([0 1 1 1-e 1-e 0+e],[0 0 1 1-e 0+e 0+e],c2);patch([0 0 1 1-e 0+e 0+e],[0 1 1 1-e 1-e 0+e],c3);plot([0 1 1 0 0],[0 0 1 1 0]);disp('Mux');
  dotprod{1..15} (15 alike) : neural/Weight Functions/dotprod
  "lz{4,3}" : Outport
      mask Display: e = 0.06;c1 = [120 230 180]/255;c2 = ([120 230 180]+0)/(256+128);c3 = ([120 230 180]+128)/(256+128);patch([0 1 1 0],[0 0 1 1],c1);patch([0 1 1 1-e 1-e 0+e],[0 0 1 1-e 0+e 0+e],c2);patch([0 0 1 1-e 0+e 0+e],[0 1 1 1-e 1-e 0+e],c3);plot([0 1 1 0 0],[0 0 1 1 0]);
  wires:
  Mux/1 -> "lz{4,3}"/1
  dotprod15/1 -> Mux/15
  "IW{4,3}(15,:)'"/1 -> dotprod15/1
  dotprod14/1 -> Mux/14
  "IW{4,3}(14,:)'"/1 -> dotprod14/1
  dotprod13/1 -> Mux/13
  "IW{4,3}(13,:)'"/1 -> dotprod13/1
  dotprod12/1 -> Mux/12
  "IW{4,3}(12,:)'"/1 -> dotprod12/1
  dotprod11/1 -> Mux/11
  "IW{4,3}(11,:)'"/1 -> dotprod11/1
  dotprod10/1 -> Mux/10
  "IW{4,3}(10,:)'"/1 -> dotprod10/1
  dotprod9/1 -> Mux/9
  "IW{4,3}(9,:)'"/1 -> dotprod9/1
  dotprod8/1 -> Mux/8
  "IW{4,3}(8,:)'"/1 -> dotprod8/1
  dotprod7/1 -> Mux/7
  "IW{4,3}(7,:)'"/1 -> dotprod7/1
  dotprod6/1 -> Mux/6
  "IW{4,3}(6,:)'"/1 -> dotprod6/1
  dotprod5/1 -> Mux/5
  "IW{4,3}(5,:)'"/1 -> dotprod5/1
  dotprod4/1 -> Mux/4
  "IW{4,3}(4,:)'"/1 -> dotprod4/1
  dotprod3/1 -> Mux/3
  "IW{4,3}(3,:)'"/1 -> dotprod3/1
  dotprod2/1 -> Mux/2
  "IW{4,3}(2,:)'"/1 -> dotprod2/1
  dotprod1/1 -> Mux/1
  "ad{4,3}"/1 -> dotprod15/2, dotprod14/2, dotprod13/2, dotprod12/2, dotprod11/2, dotprod10/2, dotprod9/2, dotprod8/2, dotprod7/2, dotprod6/2, dotprod5/2, dotprod4/2, dotprod3/2, dotprod2/2, dotprod1/2
  "IW{4,3}(1,:)'"/1 -> dotprod1/1

== system AFC_FFNN_trainscg_15_15_15_15_15_Nor_July_15_RepCont/Air Fuel Control Model 1/Feed-Forward Neural Network/Layer 5/Delays 1 ==
  "p{5}" : Inport  PortDimensions=15
      mask Display: e = 0.06;c1 = [120 230 180]/255;c2 = ([120 230 180]+0)/(256+128);c3 = ([120 230 180]+128)/(256+128);patch([0 1 1 0],[0 0 1 1],c1);patch([0 1 1 1-e 1-e 0+e],[0 0 1 1-e 0+e 0+e],c2);patch([0 0 1 1-e 0+e 0+e],[0 1 1 1-e 1-e 0+e],c3);plot([0 1 1 0 0],[0 0 1 1 0]);
  mux : Mux  Inputs=1
      mask Display: e = 0.06;c1 = [120 150 230]/255;c2 = ([120 150 230]+0)/383;c3 = ([120 150 230]+128)/383;patch([0 1 1 0],[0 0 1 1],c1);patch([0 1 1 1-e 1-e 0+e],[0 0 1 1-e 0+e 0+e],c2);patch([0 0 1 1-e 0+e 0+e],[0 1 1 1-e 1-e 0+e],c3);plot([0 1 1 0 0],[0 0 1 1 0]);disp('Mux')
  "pd{5,4}" : Outport
      mask Display: e = 0.06;c1 = [120 230 180]/255;c2 = ([120 230 180]+0)/(256+128);c3 = ([120 230 180]+128)/(256+128);patch([0 1 1 0],[0 0 1 1],c1);patch([0 1 1 1-e 1-e 0+e],[0 0 1 1-e 0+e 0+e],c2);patch([0 0 1 1-e 0+e 0+e],[0 1 1 1-e 1-e 0+e],c3);plot([0 1 1 0 0],[0 0 1 1 0]);
  wires:
  mux/1 -> "pd{5,4}"/1
  "p{5}"/1 -> mux/1
